simulink model "acc_paper_baseline"  (R2024a)
settings: Solver=FixedStepDiscrete  StartTime=0.0  StopTime=30  FixedStep=0.02  RelTol=1e-3
model workspace (MAT data in the model file):
  ego0 = [0; 16.6666666667; 0; 2146.49758775; 1]
  power0 = [0.121482339562; 0; 4]
  sceneInput = timeseries
  sceneInput.Name = 'unnamed'
  sceneInput.DataInfo = tsdata.datametadata
  sceneInput.DataInfo.Interpolation = tsdata.interpolation
  sceneInput.DataInfo.Interpolation.Fhandle : function handle (value not decoded)
  sceneInput.DataInfo.Interpolation.Name = 'linear'
  sceneInput.TimeInfo = tsdata.timemetadata
  sceneInput.TimeInfo.Length = 1501
  sceneInput.TimeInfo.DuplicateTimes = 0
  sceneInput.TimeInfo.Time_ = [0 0.02 0.04 0.06 0.08 0.1 0.12 0.14 0.16 0.18 0.2 0.22 ... (1501 elements, 1501x1)]
  sceneInput.TimeInfo.Initialized = 1
  sceneInput.QualityInfo = tsdata.qualmetadata
  sceneInput.Data_ = [16.6666666667 16.6666666667 16.6666666667 16.6666666667 16.6666666667 16.6666666667 16.6666666667 16.6666666667 16.6666666667 16.6666666667 16.6666666667 16.6666666667 ... (6004 elements, 1501x4)]
libraries: acc_control_lib x1
settings Model: Creator=26401  LastModifiedBy=26401

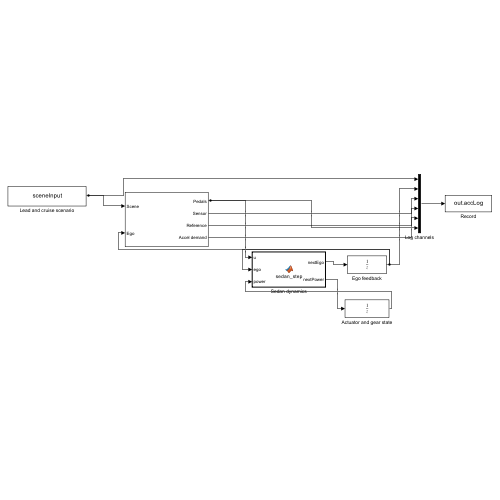
[thumbnail: Simulink's stored preview of the top-level diagram]
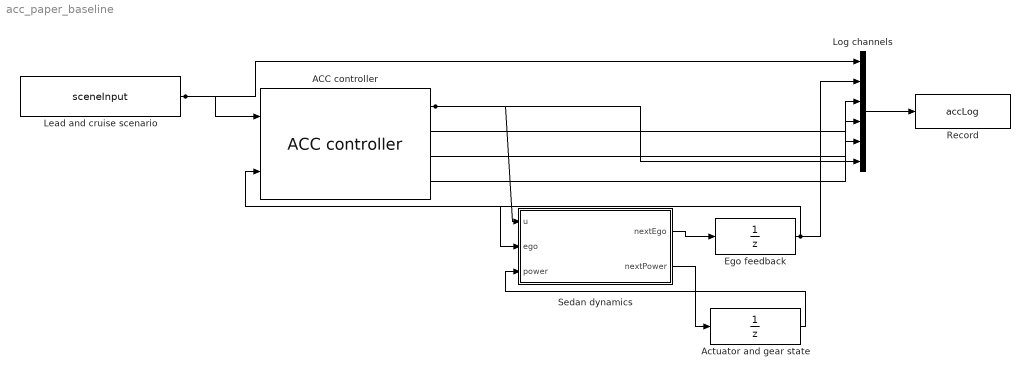
== system acc_paper_baseline ==
  ACC controller : acc_control_lib/ACC controller  SystemSampleTime=-1  VariantActivationTime=update diagram  AllowFlexibleInterface=on  Latency=0  AutoFrameSizeCalculation=off
  Actuator and gear state : UnitDelay  InitialCondition=power0  SampleTime=0.02  HasFrameUpgradeWarning=on
  Ego feedback : UnitDelay  InitialCondition=ego0  SampleTime=0.02  HasFrameUpgradeWarning=on
  Lead and cruise scenario : FromWorkspace  VariableName=sceneInput  SampleTime=0.02  OutputAfterFinalValue=Holding final value
  Log channels : Mux  Inputs=6
  Record : ToWorkspace  VariableName=accLog  SaveFormat=Timeseries  SampleTime=-1
  Sedan dynamics : MATLAB Function  TreatAsAtomicUnit=on
  wires:
  Lead and cruise scenario/1 -> ACC controller/1, Log channels/1
  Ego feedback/1 -> ACC controller/2, Sedan dynamics/2(ego), Log channels/2
  ACC controller/1 -> Sedan dynamics/1(u), Log channels/6
  Actuator and gear state/1 -> Sedan dynamics/3(power)
  Sedan dynamics/1(nextEgo) -> Ego feedback/1
  Sedan dynamics/2(nextPower) -> Actuator and gear state/1
  ACC controller/2 -> Log channels/3
  ACC controller/3 -> Log channels/4
  ACC controller/4 -> Log channels/5
  Log channels/1 -> Record/1

== matlab function acc_paper_baseline/Sedan dynamics ==
  data: u input; nextEgo output; ego input; power input; nextPower output
function [nextEgo,nextPower] = sedan_step(u,ego,power)
% Forward vehicle model. Both state vectors are delayed one tick in Simulink.
Ts = 0.02;
throttle = power(1)+(1-exp(-Ts/0.25))*(u(1)-power(1));
pressure = power(2)+(1-exp(-Ts/0.08))*(u(2)-power(2));
rearPressure = min(pressure,2) + 0.30*max(pressure-2,0);
brakeForce = 2*(350*pressure+200*rearPressure)/0.304;
[loss,traction,mass] = baseline_forces(ego(2),ego(4),ego(5));
net = (throttle*traction-brakeForce-loss)/mass;
v = max(ego(2)+Ts*net,0);
a = (v-ego(2))/Ts;
s = ego(1) + Ts*(v+ego(2))/2;
[rpm,ratio,gear] = baseline_gear(v,power(3));
nextEgo = [s;v;a;rpm;ratio];
nextPower = [throttle;pressure;gear];
end
